simulink model "Y3Tiltrotor_sim3_INDI"  (R2025a)
settings: Solver=ode4  StartTime=0.0  StopTime=70  FixedStep=uavParam.sampleTime  RelTol=1e-3
PreLoadFcn:
  | filepath  = fileparts(get_param(bdroot, 'FileName'))
  | cd(filepath);
InitFcn:
  | Init_sim_INDI;
values from neighbouring files (symbols this model uses):
  control = struct    [Init_sim_INDI.m]
  env = struct    [InitData.m]
  flightState = struct    [Init_sim_INDI.m]
  FWSpeed0 = 15    [Init_sim_INDI.m]
  k_lpf_p = 50    [Init_sim_INDI.m]
  k_lpf_q = 80    [Init_sim_INDI.m]
  k_lpf_r = 5    [Init_sim_INDI.m]
  k_lpf_u = 10    [Init_sim_INDI.m]
  k_lpf_v = 1    [Init_sim_INDI.m]
  k_lpf_w = 50    [Init_sim_INDI.m]
  k_p = 5    [Init_sim_INDI.m]
  k_q = 20    [Init_sim_INDI.m]
  k_r = 1.5    [Init_sim_INDI.m]
  k_u = 0.5    [Init_sim_INDI.m]
  k_v = 0.5    [Init_sim_INDI.m]
  k_w = 2    [Init_sim_INDI.m]
  uavParam = struct    [InitData.m]
undefined symbols (not defined in the file or in its folder): ControlSampleTime, F, Light, MIL, Newton, Raphson
libraries: slpidlib x28, SignalEditorBlockLib x12, simulink x6, aerolibtransform2 x3, sharedtransform x3, robotcorelib x3, matrix_library x3, aerolibasang x2, aerolibutil x2, aerolibwind2 x2, shared6dof x1, aerolibatmos2 x1
(part 3 of 7)

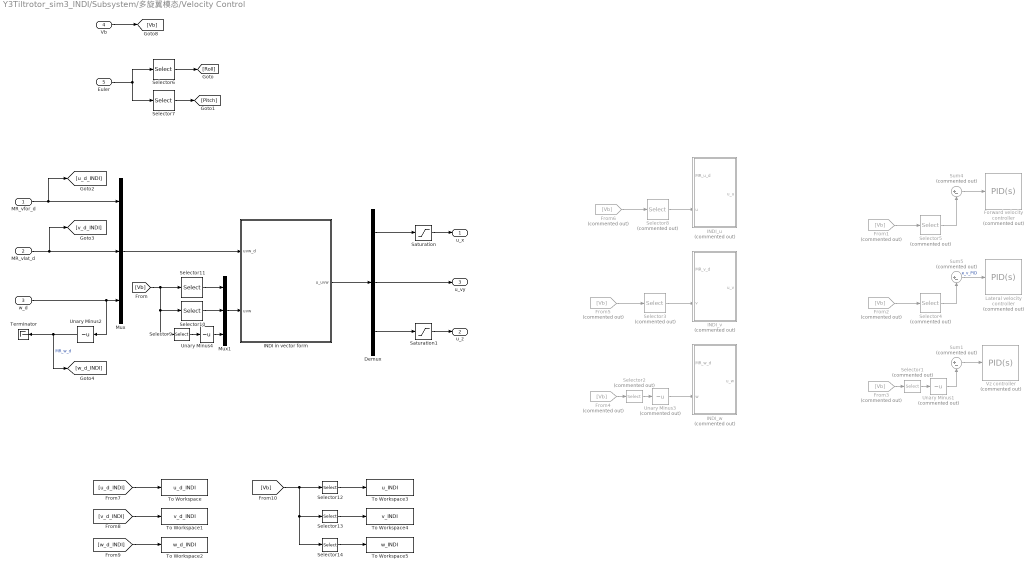
== system Y3Tiltrotor_sim3_INDI/Subsystem/多旋翼模态/Velocity Control ==
  MR_vfor_d : Inport
  MR_vlat_d : Inport  Port=2
  w_d : Inport  Port=3
  Vb : Inport  Port=4
  Euler : Inport  Port=5
  Demux : Demux  Outputs=3
  Forward velocity controller : slpidlib/PID Controller  Commented=on  Controller=PID  Form=Parallel  TimeDomain=Continuous-time  UseExternalTs=off  SampleTime=-1  IntegratorMethod=Forward Euler  FilterMethod=Forward Euler  ControllerParametersSource=internal  P=control.MR.vx_P  I=control.MR.vx_I  UseKiTs=off  D=control.MR.vx_D  UseExternalDerivativeSource=off  N=100  UseFilter=on  TunerSelectOption=Transfer Function Based (PID Tuner App)  InitialConditionSource=internal  InitialConditionForIntegrator=0  InitialConditionForFilter=0  DifferentiatorICPrevScaledInput=0  ExternalReset=none  TrackingMode=off  Kt=1  LimitOutput=off  SatLimitsSource=internal  UpperSaturationLimit=2  LowerSaturationLimit=-2  LinearizeAsGain=on  AntiWindupMode=none  Kb=1  LimitIntegrator=off  UpperIntegratorSaturationLimit=0.2  LowerIntegratorSaturationLimit=-0.2  POutMin=[]  POutMax=[]  IOutMin=[]  IOutMax=[]  DOutMin=[]  DOutMax=[]  NOutMin=[]  NOutMax=[]  SumOutMin=[]  SumOutMax=[]  SaturationOutMin=[]  SaturationOutMax=[]  PParamMin=[]  PParamMax=[]  IParamMin=[]  IParamMax=[]  DParamMin=[]  DParamMax=[]  NParamMin=[]  NParamMax=[]  KbParamMin=[]  KbParamMax=[]  KtParamMin=[]  KtParamMax=[]  KbOutMin=[]  KbOutMax=[]  KtOutMin=[]  KtOutMax=[]  IntegratorOutMin=[]  IntegratorOutMax=[]  FilterOutMin=[]  FilterOutMax=[]  SumI1OutMin=[]  SumI1OutMax=[]  SumI2OutMin=[]  SumI2OutMax=[]  SumI3OutMin=[]  SumI3OutMax=[]  SumI4OutMin=[]  SumI4OutMax=[]  SumDOutMin=[]  SumDOutMax=[]  DifferentiatorOutMin=[]  DifferentiatorOutMax=[]  FilterDiffOutCoefMin=[]  FilterDiffOutCoefMax=[]  ReciprocalOutMin=[]  ReciprocalOutMax=[]  SumDenOutMin=[]  SumDenOutMax=[]  SumNumOutMin=[]  SumNumOutMax=[]  DivideOutMin=[]  DivideOutMax=[]  UdiffTsProdOutMin=[]  UdiffTsProdOutMax=[]  NTsProdOutMin=[]  NTsProdOutMax=[]  UintegralTsProdOutMin=[]  UintegralTsProdOutMax=[]  UngainTsProdOutMin=[]  UngainTsProdOutMax=[]  ClampingZeroOutDataTypeStr=Inherit: Inherit via back propagation  ClampingZeroOutMin=[]  ClampingZeroOutMax=[]  FilterDenConstantOutDataTypeStr=Inherit: Inherit via back propagation  FilterDenConstantOutMin=[]  FilterDenConstantOutMax=[]  PCopyOutDataTypeStr=Inherit: Inherit via back propagation  PCopyOutMin=[]  PCopyOutMax=[]  NCopyOutDataTypeStr=Inherit: Inherit via back propagation  NCopyOutMin=[]  NCopyOutMax=[]  IntegratorContinuousStateAttributes=''  IntegratorStateMustResolveToSignalObject=off  IntegratorRTWStateStorageClass=Auto  FilterContinuousStateAttributes=''  FilterStateMustResolveToSignalObject=off  FilterRTWStateStorageClass=Auto  ParallelPVariant=InternalParameters  IdealPVariant=Disabled  IVariant=InternalParameters  DVariant=InternalParameters  IntegratorVariant=Continuous  SatVariant=Disabled  AWVariant=Passthrough  PCopyVariant=Disabled  TRVariant=Disabled  FdbkBlocksVariant=Forward  IdealPFdbkVariant=Disabled  SatFdbkVariant=Disabled  DerivativeFilterVariant=ContFilter  NVariant=InternalParameters  NCopyVariant=Disabled  FilterICVariant=InternalICsFilter  IntegratorICVariant=InternalICs  ExternalResetVariant=Disabled  TRSumVariant=Passthrough  SumFdbkVariant=Disabled  SumVariant=Sum_PID  TsampFilterVariant=InternalTs  TsampNgainVariant=Passthrough  TsampIntegralVariant=Disabled_SignalSpec  ExternalSaturationOutDataTypeStr=Inherit: Same as second input  DerivativeSourceVariant=ErrorSignal  PreIntVariant=InternalPreInt
  From{1..6} (6 alike) : From  Commented=on  GotoTag=Vb
  INDI in vector form : Subsystem
  INDI_u : Subsystem  Commented=on
  INDI_v : Subsystem  Commented=on
  INDI_w : Subsystem  Commented=on
  "Lateral velocity controller " : slpidlib/PID Controller  Commented=on  Controller=PID  Form=Parallel  TimeDomain=Continuous-time  UseExternalTs=off  SampleTime=-1  IntegratorMethod=Forward Euler  FilterMethod=Forward Euler  ControllerParametersSource=internal  P=control.MR.vy_P  I=control.MR.vy_I  UseKiTs=off  D=control.MR.vy_D  UseExternalDerivativeSource=off  N=100  UseFilter=on  TunerSelectOption=Transfer Function Based (PID Tuner App)  InitialConditionSource=internal  InitialConditionForIntegrator=0  InitialConditionForFilter=0  DifferentiatorICPrevScaledInput=0  ExternalReset=none  TrackingMode=off  Kt=1  LimitOutput=off  SatLimitsSource=internal  UpperSaturationLimit=control.maxRoll  LowerSaturationLimit=control.minRoll  LinearizeAsGain=on  AntiWindupMode=none  Kb=1  LimitIntegrator=off  UpperIntegratorSaturationLimit=inf  LowerIntegratorSaturationLimit=-inf  POutMin=[]  POutMax=[]  IOutMin=[]  IOutMax=[]  DOutMin=[]  DOutMax=[]  NOutMin=[]  NOutMax=[]  SumOutMin=[]  SumOutMax=[]  SaturationOutMin=[]  SaturationOutMax=[]  PParamMin=[]  PParamMax=[]  IParamMin=[]  IParamMax=[]  DParamMin=[]  DParamMax=[]  NParamMin=[]  NParamMax=[]  KbParamMin=[]  KbParamMax=[]  KtParamMin=[]  KtParamMax=[]  KbOutMin=[]  KbOutMax=[]  KtOutMin=[]  KtOutMax=[]  IntegratorOutMin=[]  IntegratorOutMax=[]  FilterOutMin=[]  FilterOutMax=[]  SumI1OutMin=[]  SumI1OutMax=[]  SumI2OutMin=[]  SumI2OutMax=[]  SumI3OutMin=[]  SumI3OutMax=[]  SumI4OutMin=[]  SumI4OutMax=[]  SumDOutMin=[]  SumDOutMax=[]  DifferentiatorOutMin=[]  DifferentiatorOutMax=[]  FilterDiffOutCoefMin=[]  FilterDiffOutCoefMax=[]  ReciprocalOutMin=[]  ReciprocalOutMax=[]  SumDenOutMin=[]  SumDenOutMax=[]  SumNumOutMin=[]  SumNumOutMax=[]  DivideOutMin=[]  DivideOutMax=[]  UdiffTsProdOutMin=[]  UdiffTsProdOutMax=[]  NTsProdOutMin=[]  NTsProdOutMax=[]  UintegralTsProdOutMin=[]  UintegralTsProdOutMax=[]  UngainTsProdOutMin=[]  UngainTsProdOutMax=[]  ClampingZeroOutDataTypeStr=Inherit: Inherit via back propagation  ClampingZeroOutMin=[]  ClampingZeroOutMax=[]  FilterDenConstantOutDataTypeStr=Inherit: Inherit via back propagation  FilterDenConstantOutMin=[]  FilterDenConstantOutMax=[]  PCopyOutDataTypeStr=Inherit: Inherit via back propagation  PCopyOutMin=[]  PCopyOutMax=[]  NCopyOutDataTypeStr=Inherit: Inherit via back propagation  NCopyOutMin=[]  NCopyOutMax=[]  IntegratorContinuousStateAttributes=''  IntegratorStateMustResolveToSignalObject=off  IntegratorRTWStateStorageClass=Auto  FilterContinuousStateAttributes=''  FilterStateMustResolveToSignalObject=off  FilterRTWStateStorageClass=Auto  ParallelPVariant=InternalParameters  IdealPVariant=Disabled  IVariant=InternalParameters  DVariant=InternalParameters  IntegratorVariant=Continuous  SatVariant=Disabled  AWVariant=Passthrough  PCopyVariant=Disabled  TRVariant=Disabled  FdbkBlocksVariant=Forward  IdealPFdbkVariant=Disabled  SatFdbkVariant=Disabled  DerivativeFilterVariant=ContFilter  NVariant=InternalParameters  NCopyVariant=Disabled  FilterICVariant=InternalICsFilter  IntegratorICVariant=InternalICs  ExternalResetVariant=Disabled  TRSumVariant=Passthrough  SumFdbkVariant=Disabled  SumVariant=Sum_PID  TsampFilterVariant=InternalTs  TsampNgainVariant=Passthrough  TsampIntegralVariant=Disabled_SignalSpec  ExternalSaturationOutDataTypeStr=Inherit: Same as second input  DerivativeSourceVariant=ErrorSignal  PreIntVariant=InternalPreInt
  Mux : Mux  Inputs=3
  Mux1 : Mux  Inputs=3
  Saturation : Saturate  UpperLimit=2  LowerLimit=-2
  Saturation1 : Saturate  UpperLimit=3  LowerLimit=0
  Selector1 : Selector  Commented=on  InputPortWidth=3  IndexOptions=Index vector (dialog)  Indices=3  OutputSizes=1
  Selector10 : Selector  InputPortWidth=3  IndexOptions=Index vector (dialog)  Indices=2  OutputSizes=1
  Selector11 : Selector  InputPortWidth=3  IndexOptions=Index vector (dialog)  Indices=1  OutputSizes=1
  Selector12 : Selector  InputPortWidth=3  IndexOptions=Index vector (dialog)  Indices=1  OutputSizes=1
  Selector13 : Selector  InputPortWidth=3  IndexOptions=Index vector (dialog)  Indices=2  OutputSizes=1
  Selector14 : Selector  InputPortWidth=3  IndexOptions=Index vector (dialog)  Indices=3  OutputSizes=1
  Selector2 : Selector  Commented=on  InputPortWidth=3  IndexOptions=Index vector (dialog)  Indices=3  OutputSizes=1
  Selector3 : Selector  Commented=on  InputPortWidth=3  IndexOptions=Index vector (dialog)  Indices=2  OutputSizes=1
  Selector4 : Selector  Commented=on  InputPortWidth=3  IndexOptions=Index vector (dialog)  Indices=2  OutputSizes=1
  Selector5 : Selector  Commented=on  InputPortWidth=3  IndexOptions=Index vector (dialog)  Indices=1  OutputSizes=1
  Selector6 : Selector  InputPortWidth=3  IndexOptions=Index vector (dialog)  Indices=1  OutputSizes=1
  Selector7 : Selector  InputPortWidth=3  IndexOptions=Index vector (dialog)  Indices=2  OutputSizes=1
  Selector8 : Selector  Commented=on  InputPortWidth=3  IndexOptions=Index vector (dialog)  Indices=1  OutputSizes=1
  Selector9 : Selector  InputPortWidth=3  IndexOptions=Index vector (dialog)  Indices=3  OutputSizes=1
  Sum1 : Sum  Commented=on  Inputs=|+-
  Sum4 : Sum  Commented=on  Inputs=|+-
  Sum5 : Sum  Commented=on  Inputs=|+-
  Terminator : Terminator
  To Workspace : ToWorkspace  VariableName=u_d_INDI  SampleTime=-1
      settings: Save2DSignal=2-D array (concatenate along first dimension)
  To Workspace1 : ToWorkspace  VariableName=v_d_INDI  SampleTime=-1
      settings: Save2DSignal=2-D array (concatenate along first dimension)
  To Workspace2 : ToWorkspace  VariableName=w_d_INDI  SampleTime=-1
      settings: Save2DSignal=2-D array (concatenate along first dimension)
  To Workspace3 : ToWorkspace  VariableName=u_INDI  SampleTime=-1
      settings: Save2DSignal=2-D array (concatenate along first dimension)
  To Workspace4 : ToWorkspace  VariableName=v_INDI  SampleTime=-1
      settings: Save2DSignal=2-D array (concatenate along first dimension)
  To Workspace5 : ToWorkspace  VariableName=w_INDI  SampleTime=-1
      settings: Save2DSignal=2-D array (concatenate along first dimension)
  Unary Minus1 : UnaryMinus  Commented=on
  Unary Minus2 : UnaryMinus
  Unary Minus3 : UnaryMinus  Commented=on
  Unary Minus4 : UnaryMinus
  Vz controller : slpidlib/PID Controller  Commented=on  Controller=PID  Form=Parallel  TimeDomain=Continuous-time  UseExternalTs=off  SampleTime=ControlSampleTime  IntegratorMethod=Forward Euler  FilterMethod=Forward Euler  ControllerParametersSource=internal  P=control.MR.vz_P  I=control.MR.vz_I  UseKiTs=off  D=control.MR.vz_D  UseExternalDerivativeSource=off  N=100  UseFilter=on  TunerSelectOption=Transfer Function Based (PID Tuner App)  InitialConditionSource=internal  InitialConditionForIntegrator=0  InitialConditionForFilter=0  DifferentiatorICPrevScaledInput=0  ExternalReset=none  TrackingMode=off  Kt=1  LimitOutput=off  SatLimitsSource=internal  UpperSaturationLimit=3  LowerSaturationLimit=0  LinearizeAsGain=on  AntiWindupMode=clamping  Kb=1  LimitIntegrator=off  UpperIntegratorSaturationLimit=inf  LowerIntegratorSaturationLimit=-inf  POutMin=[]  POutMax=[]  IOutMin=[]  IOutMax=[]  DOutMin=[]  DOutMax=[]  NOutMin=[]  NOutMax=[]  SumOutMin=[]  SumOutMax=[]  SaturationOutMin=[]  SaturationOutMax=[]  PParamMin=[]  PParamMax=[]  IParamMin=[]  IParamMax=[]  DParamMin=[]  DParamMax=[]  NParamMin=[]  NParamMax=[]  KbParamMin=[]  KbParamMax=[]  KtParamMin=[]  KtParamMax=[]  KbOutMin=[]  KbOutMax=[]  KtOutMin=[]  KtOutMax=[]  IntegratorOutMin=[]  IntegratorOutMax=[]  FilterOutMin=[]  FilterOutMax=[]  SumI1OutMin=[]  SumI1OutMax=[]  SumI2OutMin=[]  SumI2OutMax=[]  SumI3OutMin=[]  SumI3OutMax=[]  SumI4OutMin=[]  SumI4OutMax=[]  SumDOutMin=[]  SumDOutMax=[]  DifferentiatorOutMin=[]  DifferentiatorOutMax=[]  FilterDiffOutCoefMin=[]  FilterDiffOutCoefMax=[]  ReciprocalOutMin=[]  ReciprocalOutMax=[]  SumDenOutMin=[]  SumDenOutMax=[]  SumNumOutMin=[]  SumNumOutMax=[]  DivideOutMin=[]  DivideOutMax=[]  UdiffTsProdOutMin=[]  UdiffTsProdOutMax=[]  NTsProdOutMin=[]  NTsProdOutMax=[]  UintegralTsProdOutMin=[]  UintegralTsProdOutMax=[]  UngainTsProdOutMin=[]  UngainTsProdOutMax=[]  ClampingZeroOutDataTypeStr=Inherit: Inherit via back propagation  ClampingZeroOutMin=[]  ClampingZeroOutMax=[]  FilterDenConstantOutDataTypeStr=Inherit: Inherit via back propagation  FilterDenConstantOutMin=[]  FilterDenConstantOutMax=[]  PCopyOutDataTypeStr=Inherit: Inherit via back propagation  PCopyOutMin=[]  PCopyOutMax=[]  NCopyOutDataTypeStr=Inherit: Inherit via back propagation  NCopyOutMin=[]  NCopyOutMax=[]  IntegratorContinuousStateAttributes=''  IntegratorStateMustResolveToSignalObject=off  IntegratorRTWStateStorageClass=Auto  FilterContinuousStateAttributes=''  FilterStateMustResolveToSignalObject=off  FilterRTWStateStorageClass=Auto  ParallelPVariant=InternalParameters  IdealPVariant=Disabled  IVariant=InternalParameters  DVariant=InternalParameters  IntegratorVariant=Continuous  SatVariant=Disabled  AWVariant=Passthrough  PCopyVariant=Disabled  TRVariant=Disabled  FdbkBlocksVariant=Forward  IdealPFdbkVariant=Disabled  SatFdbkVariant=Disabled  DerivativeFilterVariant=ContFilter  NVariant=InternalParameters  NCopyVariant=Disabled  FilterICVariant=InternalICsFilter  IntegratorICVariant=InternalICs  ExternalResetVariant=Disabled  TRSumVariant=Passthrough  SumFdbkVariant=Disabled  SumVariant=Sum_PID  TsampFilterVariant=InternalTs  TsampNgainVariant=Passthrough  TsampIntegralVariant=Disabled_SignalSpec  ExternalSaturationOutDataTypeStr=Inherit: Same as second input  DerivativeSourceVariant=ErrorSignal  PreIntVariant=InternalPreInt
  u_x : Outport
  u_z : Outport  Port=2
  u_vy : Outport  Port=3
  wires:
  Unary Minus1/1 -> Sum1/2
  Selector1/1 -> Unary Minus1/1
  Vb/1 -> [Vb]
  From3/1 -> Selector1/1
  w_d/1 -> Mux/3, Unary Minus2/1
  Sum1/1 -> Vz controller/1
  Euler/1 -> Selector6/1, Selector7/1
  Selector7/1 -> [Pitch]
  Selector6/1 -> [Roll]
  Saturation/1 -> u_x/1
  Saturation1/1 -> u_z/1
  Unary Minus2/1 -> [w_d_INDI], Terminator/1  "MR_w_d"
  Selector4/1 -> Sum5/2
  From2/1 -> Selector4/1
  Sum5/1 -> "Lateral velocity controller "/1  "e_v_PID"
  Sum4/1 -> Forward velocity controller/1
  From1/1 -> Selector5/1
  Selector5/1 -> Sum4/2
  INDI in vector form/1(u_uvw) -> Demux/1
  Mux1/1 -> INDI in vector form/2(uvw)
  Mux/1 -> INDI in vector form/1(uvw_d)
  From6/1 -> Selector8/1
  Selector8/1 -> INDI_u/2(u)
  Selector3/1 -> INDI_v/2(v)
  From5/1 -> Selector3/1
  Unary Minus3/1 -> INDI_w/2(w)
  Selector2/1 -> Unary Minus3/1
  From4/1 -> Selector2/1
  MR_vfor_d/1 -> [u_d_INDI], Mux/1
  MR_vlat_d/1 -> [v_d_INDI], Mux/2
  Selector9/1 -> Unary Minus4/1
  [Vb] -> Selector11/1, Selector10/1, Selector9/1
  Selector11/1 -> Mux1/1
  Selector10/1 -> Mux1/2
  Unary Minus4/1 -> Mux1/3
  Demux/1 -> Saturation/1
  Demux/2 -> u_vy/1
  Demux/3 -> Saturation1/1
  [u_d_INDI] -> To Workspace/1
  [v_d_INDI] -> To Workspace1/1
  [w_d_INDI] -> To Workspace2/1
  [Vb] -> Selector13/1, Selector14/1, Selector12/1
  Selector12/1 -> To Workspace3/1
  Selector13/1 -> To Workspace4/1
  Selector14/1 -> To Workspace5/1

== system Y3Tiltrotor_sim3_INDI/Subsystem/混控器/固定翼混控 ==
  FlightMode : Inport
  "FixedwingControlOutput " : Inport  Port=2
  Merge : Merge  Inputs=4
  Switch Case : SwitchCase  CaseConditions={flightState.Hover, flightState.Transition, flightState.FixedWing,flightState.BackTransition}  ShowDefaultCase=off
  固定翼模态混控 : Subsystem
  旋翼模态混控 : Subsystem
  toMultirotorMixer : Outport
  FixedwingCtrlSurface : Outport  Port=2
  wires:
  "FixedwingControlOutput "/1 -> 固定翼模态混控/1("FixedwingControlOutput ")
  固定翼模态混控/1(toMultirotorMixer) -> toMultirotorMixer/1
  FlightMode/1 -> Switch Case/1
  Merge/1 -> FixedwingCtrlSurface/1
  固定翼模态混控/2(FixedwingCtrlSurface) -> Merge/3
  Switch Case/3 -> 固定翼模态混控/Action
  旋翼模态混控/1(FixedwingCtrlSurface) -> Merge/1
  Switch Case/1 -> 旋翼模态混控/Action

== system Y3Tiltrotor_sim3_INDI/Subsystem/混控器/多旋翼混控 ==
  States : Inport
  "MultirotorControlOutput " : Inport  Port=2
  FlightMode : Inport  Port=3
  toMultirotorMixer : Inport  Port=4
  Actuator To Voltage : Subsystem
  Merge : Merge  Inputs=4
  Switch Case : SwitchCase  CaseConditions={flightState.Hover, flightState.Transition, flightState.FixedWing,flightState.BackTransition}  ShowDefaultCase=off
  固定翼模态混控 : Subsystem
  旋翼模态混控 : Subsystem
  MultirotorActuator : Outport
  wires:
  toMultirotorMixer/1 -> 固定翼模态混控/1(toMultirotorMixer)
  固定翼模态混控/1(MultirotorActuator) -> Merge/3
  FlightMode/1 -> Switch Case/1
  Switch Case/3 -> 固定翼模态混控/Action
  Switch Case/1 -> 旋翼模态混控/Action
  "MultirotorControlOutput "/1 -> 旋翼模态混控/1("MultirotorControlOutput ")
  旋翼模态混控/1(MultirotorActuator) -> Merge/1
  Actuator To Voltage/1(To PWM) -> MultirotorActuator/1
  Merge/1 -> Actuator To Voltage/1(Motor Commands)
  States/1 -> 旋翼模态混控/2(states)

== system Y3Tiltrotor_sim3_INDI/Y3 Tiltrotor Aircraft Model/Subsystem/Aerodynamic Forces and Moments ==
  note: FIMI Manta飞行器气动力和力矩的计算需要参考飞翼布局的飞行器，它只有升降副翼，没有尾翼。
  CtrlSurfaces : Inport
  Wind_e : Inport  Port=2
  UAV State : Inport  Port=3
  Bus Selector2 : BusSelector  OutputSignals=DCMbe,Ve,Xe
  Compute Air Data : Subsystem  TreatAsAtomicUnit=on  VariantControl=use_aerospace_blocks == 1
  Compute Body Frame Aerodynamic Forces and Moments : Subsystem
  Compute Rho : Subsystem
  RL2B * Vw : Product  Multiplication=Matrix(*)  InputSameDT=on  SaturateOnIntegerOverflow=on  OutDataTypeStr=Inherit: Same as first input
  Vair : Sum  Inputs=+-  InputSameDT=on  SaturateOnIntegerOverflow=on  OutDataTypeStr=Inherit: Same as first input
  AirData : Outport  VectorParamsAs1DForOutWhenUnconnected=off
  F_aero : Outport  Port=2  VectorParamsAs1DForOutWhenUnconnected=off
  M_aero : Outport  Port=3  VectorParamsAs1DForOutWhenUnconnected=off
  wires:
  Bus Selector2/2 -> Vair/1  "<Ve>"
  UAV State/1 -> Bus Selector2/1
  Wind_e/1 -> Vair/2
  Compute Air Data/1(AirData) -> AirData/1, Compute Body Frame Aerodynamic Forces and Moments/1(AirData)
  RL2B * Vw/1 -> Compute Air Data/1(Vb)
  Compute Rho/1(Rho) -> Compute Air Data/2(Rho)
  Vair/1 -> RL2B * Vw/2
  Bus Selector2/3 -> Compute Rho/1(Xe)  "<Xe>"
  Bus Selector2/1 -> RL2B * Vw/1  "<DCMbe>"
  CtrlSurfaces/1 -> Compute Body Frame Aerodynamic Forces and Moments/2(CtrlSurfaces)
  Compute Body Frame Aerodynamic Forces and Moments/1(F_b) -> F_aero/1
  Compute Body Frame Aerodynamic Forces and Moments/2(M_b) -> M_aero/1

== system Y3Tiltrotor_sim3_INDI/Y3 Tiltrotor Aircraft Model/Subsystem/Gravity ==
  DCM_be : Inport
  Constant : Constant  Value=[0 0 uavParam.aero.g]'
  Gain : Gain  Gain=uavParam.geom.mass
  Matrix Multiply : Product  Multiplication=Matrix(*)
  F_g : Outport
  wires:
  Matrix Multiply/1 -> Gain/1
  Constant/1 -> Matrix Multiply/2
  DCM_be/1 -> Matrix Multiply/1
  Gain/1 -> F_g/1

== system Y3Tiltrotor_sim3_INDI/Y3 Tiltrotor Aircraft Model/Subsystem/GroundModel1 ==
  UavState : Inport
  "TerrainZ " : Inport  Port=2
  Bus Selector : BusSelector  OutputSignals=pqr,Xe,Ve,Euler,DCMbe
  Direction Cosine Matrix to Quaternions : sharedtransform/Direction Cosine Matrix  to Quaternions  aMode=aMode  action=None  tolerance=eps(2)
  Direction Cosine Matrix to Quaternions1 : sharedtransform/Direction Cosine Matrix  to Quaternions  aMode=aMode  action=None  tolerance=eps(2)
  Euler to DCM : aerolibtransform2/Wind Angles to  Direction Cosine Matrix
  Gain : Gain  Gain=[0 0 9.8]
  Ground Model New : Subsystem
  ModelParam.uavMass : Constant  Value=uavParam.geom.mass
  OnGroundFaceup : Subsystem
  Product : Product  Multiplication=Matrix(*)
  Quaternion Inverse : aerolibutil/Quaternion Inverse
  Quaternion Multiplication : aerolibutil/Quaternion Multiplication
  F_Ground : Outport  VectorParamsAs1DForOutWhenUnconnected=off
  M_Ground : Outport  Port=2  VectorParamsAs1DForOutWhenUnconnected=off
  wires:
  "TerrainZ "/1 -> Ground Model New/6(TerrainZ)
  Ground Model New/2(M1) -> M_Ground/1  "Mb"
  Product/1 -> F_Ground/1  "Fb"
  Quaternion Multiplication/1 -> Ground Model New/5(Quet)
  Quaternion Inverse/1 -> Quaternion Multiplication/1
  Direction Cosine Matrix to Quaternions1/1 -> Quaternion Inverse/1
  Euler to DCM/1 -> Direction Cosine Matrix to Quaternions1/1
  OnGroundFaceup/1(y) -> Euler to DCM/1
  Direction Cosine Matrix to Quaternions/1 -> Quaternion Multiplication/2
  Ground Model New/1(F1) -> Product/2
  UavState/1 -> Bus Selector/1
  ModelParam.uavMass/1 -> Gain/1
  Gain/1 -> Ground Model New/1(mg)
  Bus Selector/5 -> Product/1, Direction Cosine Matrix to Quaternions/1  "<DCMbe>"
  Bus Selector/4 -> OnGroundFaceup/1(Eular(rad))  "<Euler>"
  Bus Selector/3 -> Ground Model New/4(Ve)  "<Ve>"
  Bus Selector/2 -> Ground Model New/3(Xe)  "<Xe>"
  Bus Selector/1 -> Ground Model New/2(wb)  "<pqr>"

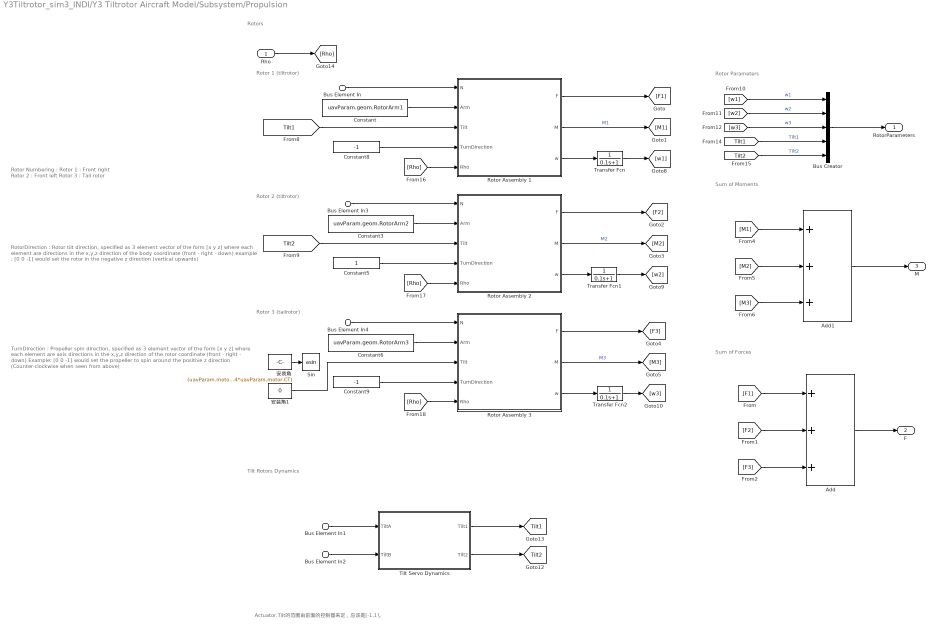
== system Y3Tiltrotor_sim3_INDI/Y3 Tiltrotor Aircraft Model/Subsystem/Propulsion ==
  note: Actuator.Tilt的范围由前面的控制器来定，应该是[-1,1]。
  note: TurnDirection : Propeller spin direction, specified as 3 element vector of the form [x y z] where each element are axis directions in the x,y,z direction of the rotor coordinate (front - right - down)
      |
      | Example: [0 0 -1] would set the propeller to spin around the positive z direction (Counter-clockwise when seen from above)
  note: RotorDirection : Rotor tilt direction, specified as 3 element vector of the form [x y z] where each element are directions in the x,y,z direction of the body coordinate (front - right - down)
      |
      | example : [0 0 -1] would set the rotor in the negative z direction (vertical upwards)
  note: Rotor Numbering :
      | Rotor 1 : Front right
      | Rotor 2 : Front left
      | Rotor 3 : Tail rotor
  note: Tilt Rotors Dynamics
  note: Sum of Moments
  note: Rotor 1
      | (tiltrotor)
  note: Rotors
  note: Rotor 2
      | (tiltrotor)
  note: Rotor 3
      | (tailrotor)
  note: Sum of Forces
  note: Rotor Parameters
  Rho : Inport
  Bus Element In : Inport  Port=2  PortName=Actuator  Element=w1
  Bus Element In1 : Inport  Port=2  PortName=Actuator  Element=Tilt1
  Bus Element In2 : Inport  Port=2  PortName=Actuator  Element=Tilt2
  Bus Element In3 : Inport  Port=2  PortName=Actuator  Element=w2
  Bus Element In4 : Inport  Port=2  PortName=Actuator  Element=w3
  Add : Sum  Inputs=+++
  Add1 : Sum  Inputs=+++
  Bus Creator : BusCreator  Inputs=5
  Constant : Constant  Value=uavParam.geom.RotorArm1
  Constant3 : Constant  Value=uavParam.geom.RotorArm2
  Constant5 : Constant
  Constant6 : Constant  Value=uavParam.geom.RotorArm3
  Constant8 : Constant  Value=-1
  Constant9 : Constant  Value=-1
  Rotor Assembly 1 : Subsystem
  Rotor Assembly 2 : Subsystem
  "Rotor Assembly 3 " : Subsystem
  Sin : Trigonometry  Operator=asin
  Tilt Servo Dynamics : Subsystem
  Transfer Fcn : TransferFcn  Denominator=[0.1 1]
  Transfer Fcn1 : TransferFcn  Denominator=[0.1 1]
  Transfer Fcn2 : TransferFcn  Denominator=[0.1 1]
  安装角 : Constant  Value=(uavParam.motor.CQ*uavParam.geom.PropRadius)/(0.24*uavParam.motor.CT)
  安装角1 : Constant  Value=0
  RotorParameters : Outport
  F : Outport  Port=2
  M : Outport  Port=3
  tag scope: Tilt1=global, Tilt2=global
  wires:
  Constant/1 -> Rotor Assembly 1/2(Arm)
  [Tilt1] -> Rotor Assembly 1/3(Tilt)
  Add/1 -> F/1
  Constant8/1 -> Rotor Assembly 1/4(TurnDirection)
  Rotor Assembly 1/1(F) -> [F1]
  Rotor Assembly 1/2(M) -> [M1]  "M1"
  Rotor Assembly 2/1(F) -> [F2]
  Constant3/1 -> Rotor Assembly 2/2(Arm)
  Constant5/1 -> Rotor Assembly 2/4(TurnDirection)
  Rotor Assembly 2/2(M) -> [M2]  "M2"
  "Rotor Assembly 3 "/1(F) -> [F3]
  Constant6/1 -> "Rotor Assembly 3 "/2(Arm)
  Constant9/1 -> "Rotor Assembly 3 "/4(TurnDirection)
  安装角/1 -> Sin/1
  "Rotor Assembly 3 "/2(M) -> [M3]  "M3"
  [F1] -> Add/1
  [F2] -> Add/2
  [F3] -> Add/3
  Add1/1 -> M/1
  [M3] -> Add1/3
  [M2] -> Add1/2
  [M1] -> Add1/1
  Rotor Assembly 1/3(w) -> Transfer Fcn/1
  Rotor Assembly 2/3(w) -> Transfer Fcn1/1
  "Rotor Assembly 3 "/3(w) -> Transfer Fcn2/1
  [w1] -> Bus Creator/1  "w1"
  [w2] -> Bus Creator/2  "w2"
  [w3] -> Bus Creator/3  "w3"
  Bus Creator/1 -> RotorParameters/1
  [Tilt1] -> Bus Creator/4  "Tilt1"
  [Tilt2] -> Bus Creator/5  "Tilt2"
  Bus Element In/1 -> Rotor Assembly 1/1(N)
  Bus Element In3/1 -> Rotor Assembly 2/1(N)
  Bus Element In4/1 -> "Rotor Assembly 3 "/1(N)
  Tilt Servo Dynamics/1(Tilt1) -> [Tilt1]
  Tilt Servo Dynamics/2(Tilt2) -> [Tilt2]
  Bus Element In1/1 -> Tilt Servo Dynamics/1(TiltA)
  Bus Element In2/1 -> Tilt Servo Dynamics/2(TiltB)
  Transfer Fcn/1 -> [w1]
  Transfer Fcn1/1 -> [w2]
  Transfer Fcn2/1 -> [w3]
  Rho/1 -> [Rho]
  [Rho] -> Rotor Assembly 1/5(Rho)
  [Tilt2] -> Rotor Assembly 2/3(Tilt)
  [Rho] -> Rotor Assembly 2/5(Rho)
  [Rho] -> "Rotor Assembly 3 "/5(Rho)
  安装角1/1 -> "Rotor Assembly 3 "/3(Tilt)

== system Y3Tiltrotor_sim3_INDI/Y3 Tiltrotor Aircraft Model/Subsystem/Weather Model_org ==
  UavState : Inport
  if Wind On : Inport  Port=2
  " Compute Norm" : Subsystem
  Add : Sum  Inputs=2
  Bus Selector : BusSelector  OutputSignals=Euler,Xe,Ve
  Constant : Constant  Value=[0 0 0]
      settings: AttributesFormatString=%<Value>
  Dryden Wind Turbulence Model : aerolibwind2/Dryden Wind Turbulence Model  (Continuous (+q -r))  units=Metric (MKS)  spec=MIL-F-8785C  model=Continuous Dryden (+q -r)  W20=env.windBase/4  Wdeg=env.windDirTurb  TurbProb=10^-2 - Light  L_high=533.4  Wingspan=uavParam.geom.span  ts=ap.apSampleTime  Seed=[23341 23342 23343 23344]  T_on=on
  Gain1 : Gain  Gain=-1
      settings: AttributesFormatString=Z to Alt
  Get Z1 : Selector  InputPortWidth=3  IndexOptions=Index vector (dialog)  Indices=[3]  OutputSizes=[(-2)]
  "Horizontal Wind Model " : aerolibwind2/Horizontal Wind Model  units=Metric (MKS)  Vw_source=Internal  Vwind=env.windBase  W_source=Internal  Wdeg=env.windDirHor
  RL2B : Subsystem
  Reduce Z Wind : Gain  Gain=[1 1 0.1]
      settings: AttributesFormatString=%<Gain>
  Rotate to E Frame : Product  Multiplication=Matrix(*)
  Switch : Switch  Criteria=u2 > Threshold  Threshold=0.3  SaturateOnIntegerOverflow=off  InputSameDT=off
  Terminator : Terminator
  Transpose : Math  Operator=transpose  SignedPower=on
  "[0, pi] Wrap Around" : Subsystem
  Wind_e : Outport  Unit=m/s  VectorParamsAs1DForOutWhenUnconnected=off
  wires:
  Bus Selector/1 -> "[0, pi] Wrap Around"/1(Euler)  "<Euler>"
  Dryden Wind Turbulence Model/2 -> Terminator/1
  Constant/1 -> Switch/3
  Get Z1/1 -> Gain1/1
  RL2B/1(RL2B) -> "Horizontal Wind Model "/1, Dryden Wind Turbulence Model/3, Transpose/1  "RECEF2B"
  Transpose/1 -> Rotate to E Frame/1
  Rotate to E Frame/1 -> Wind_e/1
  Switch/1 -> Rotate to E Frame/2
  Dryden Wind Turbulence Model/1 -> Reduce Z Wind/1
  " Compute Norm"/1(V) -> Dryden Wind Turbulence Model/2
  Gain1/1 -> Dryden Wind Turbulence Model/1
  "Horizontal Wind Model "/1 -> Add/2
  Reduce Z Wind/1 -> Add/1
  Add/1 -> Switch/1
  if Wind On/1 -> Switch/2
  "[0, pi] Wrap Around"/1(Wrapped) -> RL2B/1(Euler)  "Euler"
  UavState/1 -> Bus Selector/1
  Bus Selector/3 -> " Compute Norm"/1(<Ve>)  "<Ve>"
  Bus Selector/2 -> Get Z1/1  "<Xe>"

== system Y3Tiltrotor_sim3_INDI/Subsystem/固定翼模态/attitude control/Turn Coordinator ==
  Roll SP : Inport
  Pitch SP : Inport  Port=2
  Airspeed : Inport  Port=3
  r : Inport  Port=4
  MATLAB Function : MATLAB Function  TreatAsAtomicUnit=on
  Sum : Sum  Inputs=|+-
  YawRate Controller : slpidlib/PID Controller  Controller=PID  Form=Parallel  TimeDomain=Discrete-time  UseExternalTs=off  SampleTime=-1  IntegratorMethod=Forward Euler  FilterMethod=Forward Euler  ControllerParametersSource=internal  P=control.FW.yawRate_P  I=control.FW.yawRate_I  UseKiTs=off  D=control.FW.yawRate_D  UseExternalDerivativeSource=off  N=100  UseFilter=on  TunerSelectOption=Transfer Function Based (PID Tuner App)  InitialConditionSource=internal  InitialConditionForIntegrator=0  InitialConditionForFilter=0  DifferentiatorICPrevScaledInput=0  ExternalReset=none  TrackingMode=off  Kt=1  LimitOutput=on  SatLimitsSource=internal  UpperSaturationLimit=1  LowerSaturationLimit=-1  LinearizeAsGain=on  AntiWindupMode=none  Kb=1  LimitIntegrator=off  UpperIntegratorSaturationLimit=inf  LowerIntegratorSaturationLimit=-inf  POutMin=[]  POutMax=[]  IOutMin=[]  IOutMax=[]  DOutMin=[]  DOutMax=[]  NOutMin=[]  NOutMax=[]  SumOutMin=[]  SumOutMax=[]  SaturationOutMin=[]  SaturationOutMax=[]  PParamMin=[]  PParamMax=[]  IParamMin=[]  IParamMax=[]  DParamMin=[]  DParamMax=[]  NParamMin=[]  NParamMax=[]  KbParamMin=[]  KbParamMax=[]  KtParamMin=[]  KtParamMax=[]  KbOutMin=[]  KbOutMax=[]  KtOutMin=[]  KtOutMax=[]  IntegratorOutMin=[]  IntegratorOutMax=[]  FilterOutMin=[]  FilterOutMax=[]  SumI1OutMin=[]  SumI1OutMax=[]  SumI2OutMin=[]  SumI2OutMax=[]  SumI3OutMin=[]  SumI3OutMax=[]  SumI4OutMin=[]  SumI4OutMax=[]  SumDOutMin=[]  SumDOutMax=[]  DifferentiatorOutMin=[]  DifferentiatorOutMax=[]  FilterDiffOutCoefMin=[]  FilterDiffOutCoefMax=[]  ReciprocalOutMin=[]  ReciprocalOutMax=[]  SumDenOutMin=[]  SumDenOutMax=[]  SumNumOutMin=[]  SumNumOutMax=[]  DivideOutMin=[]  DivideOutMax=[]  UdiffTsProdOutMin=[]  UdiffTsProdOutMax=[]  NTsProdOutMin=[]  NTsProdOutMax=[]  UintegralTsProdOutMin=[]  UintegralTsProdOutMax=[]  UngainTsProdOutMin=[]  UngainTsProdOutMax=[]  ClampingZeroOutDataTypeStr=Inherit: Inherit via back propagation  ClampingZeroOutMin=[]  ClampingZeroOutMax=[]  FilterDenConstantOutDataTypeStr=Inherit: Inherit via back propagation  FilterDenConstantOutMin=[]  FilterDenConstantOutMax=[]  PCopyOutDataTypeStr=Inherit: Inherit via back propagation  PCopyOutMin=[]  PCopyOutMax=[]  NCopyOutDataTypeStr=Inherit: Inherit via back propagation  NCopyOutMin=[]  NCopyOutMax=[]  IntegratorContinuousStateAttributes=''  IntegratorStateMustResolveToSignalObject=off  IntegratorRTWStateStorageClass=Auto  FilterContinuousStateAttributes=''  FilterStateMustResolveToSignalObject=off  FilterRTWStateStorageClass=Auto  ParallelPVariant=InternalParameters  IdealPVariant=Disabled  IVariant=InternalParameters  DVariant=InternalParameters  IntegratorVariant=Discrete  SatVariant=Enabled  AWVariant=Passthrough  PCopyVariant=Disabled  TRVariant=Disabled  FdbkBlocksVariant=Forward  IdealPFdbkVariant=Disabled  SatFdbkVariant=Disabled  DerivativeFilterVariant=ForwardEulerFilter  NVariant=InternalParameters  NCopyVariant=Disabled  FilterICVariant=InternalICsFilter  IntegratorICVariant=InternalICs  ExternalResetVariant=Disabled  TRSumVariant=Passthrough  SumFdbkVariant=Disabled  SumVariant=Sum_PID  TsampFilterVariant=InternalTs  TsampNgainVariant=Passthrough  TsampIntegralVariant=Disabled_SignalSpec  ExternalSaturationOutDataTypeStr=Inherit: Same as second input  DerivativeSourceVariant=ErrorSignal  PreIntVariant=InternalPreInt
  Tau_z : Outport
  wires:
  Roll SP/1 -> MATLAB Function/1(rollSP)
  Pitch SP/1 -> MATLAB Function/2(pitchSP)
  Airspeed/1 -> MATLAB Function/3(airSpeed)
  Sum/1 -> YawRate Controller/1
  YawRate Controller/1 -> Tau_z/1  "Tau_z"
  r/1 -> Sum/2  "r"
  MATLAB Function/1(rSP) -> Sum/1  "FW_r_d"

== system Y3Tiltrotor_sim3_INDI/Subsystem/固定翼模态/高度-速度控制/定速模式 ==
  Height_d : Inport
  Xe : Inport  Port=2
  Ve : Inport  Port=3
  Manual Vz_d : Inport  Port=4
  Manual : Inport  Port=5
  FW_Airspeed_d : Inport  Port=6
  V_ref : Inport  Port=7
  Airspeed : Inport  Port=8
  gamma : Inport  Port=9
  CoupledControl : Inport  Port=10
  Action Port : ActionPort  ActionPortLabel=case [ 2 ]:
  Subsystem1 : Subsystem
  Switch : Switch  Criteria=u2 > Threshold  SaturateOnIntegerOverflow=off  InputSameDT=off
  Switch1 : Switch  Criteria=u2 > Threshold  SaturateOnIntegerOverflow=off  InputSameDT=off
  TECS : Subsystem
  airspeed control : Subsystem
  Pitch_d_spe : Outport
  Thrust_spe : Outport  Port=2
  wires:
  Height_d/1 -> Subsystem1/3(Height_d), TECS/2(h_d)
  Xe/1 -> TECS/3(Xe), Subsystem1/5(Xe)
  FW_Airspeed_d/1 -> TECS/4(Airspeed_d), airspeed control/2(Airspeed_d)
  Airspeed/1 -> TECS/6(Airspeed), airspeed control/4(Airspeed)
  gamma/1 -> TECS/7(gamma)
  TECS/2(Throttle) -> Switch/1
  CoupledControl/1 -> Switch/2, Switch1/2
  TECS/1(Theta_d) -> Switch1/1
  Switch1/1 -> Pitch_d_spe/1
  Switch/1 -> Thrust_spe/1
  airspeed control/1(Throttle) -> Switch/3
  Subsystem1/1(Pitch_d_alt) -> Switch1/3
  Ve/1 -> Subsystem1/2(Ve)
  Manual Vz_d/1 -> Subsystem1/4(Manual Vz_d)
  Manual/1 -> airspeed control/1(Manual), TECS/1(Manual), Subsystem1/1(Manual)
  V_ref/1 -> airspeed control/3(V_ref), TECS/5(V_ref)

== system Y3Tiltrotor_sim3_INDI/Subsystem/固定翼模态/高度-速度控制/定高模式 ==
  FW_Thrust_sta : Inport
  Manual : Inport  Port=2
  Manual Vz_d : Inport  Port=3
  Ve : Inport  Port=4
  Height_d : Inport  Port=5
  Xe : Inport  Port=6
  Action Port : ActionPort  ActionPortLabel=case [ 1 ]:
  Gain : Gain  Gain=-1
  PID Controller1 : slpidlib/PID Controller  Controller=PID  Form=Parallel  TimeDomain=Continuous-time  UseExternalTs=off  SampleTime=ControlSampleTime  IntegratorMethod=Forward Euler  FilterMethod=Forward Euler  ControllerParametersSource=internal  P=control.FW.vz_P  I=control.FW.vz_I  UseKiTs=off  D=control.FW.vz_D  UseExternalDerivativeSource=off  N=100  UseFilter=on  TunerSelectOption=Transfer Function Based (PID Tuner App)  InitialConditionSource=internal  InitialConditionForIntegrator=0  InitialConditionForFilter=0  DifferentiatorICPrevScaledInput=0  ExternalReset=none  TrackingMode=off  Kt=1  LimitOutput=on  SatLimitsSource=internal  UpperSaturationLimit=control.maxPitch  LowerSaturationLimit=control.minPitch  LinearizeAsGain=on  AntiWindupMode=clamping  Kb=1  LimitIntegrator=off  UpperIntegratorSaturationLimit=inf  LowerIntegratorSaturationLimit=-inf  POutMin=[]  POutMax=[]  IOutMin=[]  IOutMax=[]  DOutMin=[]  DOutMax=[]  NOutMin=[]  NOutMax=[]  SumOutMin=[]  SumOutMax=[]  SaturationOutMin=[]  SaturationOutMax=[]  PParamMin=[]  PParamMax=[]  IParamMin=[]  IParamMax=[]  DParamMin=[]  DParamMax=[]  NParamMin=[]  NParamMax=[]  KbParamMin=[]  KbParamMax=[]  KtParamMin=[]  KtParamMax=[]  KbOutMin=[]  KbOutMax=[]  KtOutMin=[]  KtOutMax=[]  IntegratorOutMin=[]  IntegratorOutMax=[]  FilterOutMin=[]  FilterOutMax=[]  SumI1OutMin=[]  SumI1OutMax=[]  SumI2OutMin=[]  SumI2OutMax=[]  SumI3OutMin=[]  SumI3OutMax=[]  SumI4OutMin=[]  SumI4OutMax=[]  SumDOutMin=[]  SumDOutMax=[]  DifferentiatorOutMin=[]  DifferentiatorOutMax=[]  FilterDiffOutCoefMin=[]  FilterDiffOutCoefMax=[]  ReciprocalOutMin=[]  ReciprocalOutMax=[]  SumDenOutMin=[]  SumDenOutMax=[]  SumNumOutMin=[]  SumNumOutMax=[]  DivideOutMin=[]  DivideOutMax=[]  UdiffTsProdOutMin=[]  UdiffTsProdOutMax=[]  NTsProdOutMin=[]  NTsProdOutMax=[]  UintegralTsProdOutMin=[]  UintegralTsProdOutMax=[]  UngainTsProdOutMin=[]  UngainTsProdOutMax=[]  ClampingZeroOutDataTypeStr=Inherit: Inherit via back propagation  ClampingZeroOutMin=[]  ClampingZeroOutMax=[]  FilterDenConstantOutDataTypeStr=Inherit: Inherit via back propagation  FilterDenConstantOutMin=[]  FilterDenConstantOutMax=[]  PCopyOutDataTypeStr=Inherit: Inherit via back propagation  PCopyOutMin=[]  PCopyOutMax=[]  NCopyOutDataTypeStr=Inherit: Inherit via back propagation  NCopyOutMin=[]  NCopyOutMax=[]  IntegratorContinuousStateAttributes=''  IntegratorStateMustResolveToSignalObject=off  IntegratorRTWStateStorageClass=Auto  FilterContinuousStateAttributes=''  FilterStateMustResolveToSignalObject=off  FilterRTWStateStorageClass=Auto  ParallelPVariant=InternalParameters  IdealPVariant=Disabled  IVariant=InternalParameters  DVariant=InternalParameters  IntegratorVariant=Continuous  SatVariant=Enabled  AWVariant=ContClampingParallel  PCopyVariant=Disabled  TRVariant=Disabled  FdbkBlocksVariant=Forward  IdealPFdbkVariant=Disabled  SatFdbkVariant=Disabled  DerivativeFilterVariant=ContFilter  NVariant=InternalParameters  NCopyVariant=Disabled  FilterICVariant=InternalICsFilter  IntegratorICVariant=InternalICs  ExternalResetVariant=Disabled  TRSumVariant=Passthrough  SumFdbkVariant=Disabled  SumVariant=Sum_PID  TsampFilterVariant=InternalTs  TsampNgainVariant=Passthrough  TsampIntegralVariant=Disabled_SignalSpec  ExternalSaturationOutDataTypeStr=Inherit: Same as second input  DerivativeSourceVariant=ErrorSignal  PreIntVariant=InternalPreInt
  Selector1 : Selector  InputPortWidth=3  IndexOptions=Index vector (dialog)  Indices=3  OutputSizes=1
  Subsystem : Subsystem
  Sum1 : Sum  Inputs=|+-
  Terminator : Terminator
  Transfer Fcn : TransferFcn  Numerator=[5]  Denominator=[1 5]
  Unary Minus1 : UnaryMinus
  Pitch_d_alt : Outport
  Thrust_alt : Outport  Port=2
  wires:
  FW_Thrust_sta/1 -> Thrust_alt/1
  Ve/1 -> Selector1/1
  Sum1/1 -> PID Controller1/1
  Selector1/1 -> Unary Minus1/1
  Gain/1 -> Terminator/1  "Vz_d"
  Transfer Fcn/1 -> Gain/1, Sum1/1
  Unary Minus1/1 -> Sum1/2
  PID Controller1/1 -> Pitch_d_alt/1
  Subsystem/1(Vz_d) -> Transfer Fcn/1
  Manual/1 -> Subsystem/1(Manual)
  Manual Vz_d/1 -> Subsystem/3(Manual Vz_d)
  Xe/1 -> Subsystem/4(Xe)
  Height_d/1 -> Subsystem/2(Height_d)

== system Y3Tiltrotor_sim3_INDI/Subsystem/固定翼模态/高度-速度控制/自稳模式 ==
  FW_Pitch_d_sta : Inport
  FW_Thrust_sta : Inport  Port=2
  Action Port : ActionPort  ActionPortLabel=case [ 0 ]:
  Pitch_d_sta : Outport
  Thrust_sta : Outport  Port=2
  wires:
  FW_Pitch_d_sta/1 -> Pitch_d_sta/1
  FW_Thrust_sta/1 -> Thrust_sta/1

== system Y3Tiltrotor_sim3_INDI/Subsystem/多旋翼模态/Multirotor XY control/Subsystem ==
  y : Inport
  Manual : Inport  Port=2
  Ch2 : Inport  Port=3
  y_ref : Inport  Port=4
  InputConditioning_altitude : Subsystem
  Merge : Merge
  Subsystem : Subsystem
  Switch Case : SwitchCase  CaseConditions={0,1}  ShowDefaultCase=off
  MR_vy_d : Outport
  wires:
  Ch2/1 -> InputConditioning_altitude/1(Ch2)
  InputConditioning_altitude/1(manual_vlat_cmd) -> Merge/2  "Manual vy_d"
  Manual/1 -> Switch Case/1
  Switch Case/2 -> InputConditioning_altitude/Action
  Subsystem/1(PID_vy_cmd) -> Merge/1  "PID_vy_d"
  Switch Case/1 -> Subsystem/Action
  Merge/1 -> MR_vy_d/1
  y_ref/1 -> Subsystem/1(y_ref)
  y/1 -> Subsystem/2(y)

== system Y3Tiltrotor_sim3_INDI/Subsystem/多旋翼模态/Multirotor XY control/Subsystem3 ==
  Manual : Inport
  Ch8 : Inport  Port=2
  x_ref : Inport  Port=3
  x : Inport  Port=4
  InputConditioning_altitude : Subsystem
  Merge : Merge
  Subsystem : Subsystem
  Switch Case : SwitchCase  CaseConditions={0,1}  ShowDefaultCase=off
  MR_vx_d : Outport
  wires:
  Merge/1 -> MR_vx_d/1
  Switch Case/1 -> Subsystem/Action
  Subsystem/1(PID_vx_cmd) -> Merge/1  "PID_vx_d"
  Switch Case/2 -> InputConditioning_altitude/Action
  Manual/1 -> Switch Case/1
  InputConditioning_altitude/1(manual_vfor_cmd) -> Merge/2  "Manual vx_d"
  Ch8/1 -> InputConditioning_altitude/1(Ch8)
  x_ref/1 -> Subsystem/1(x_ref)
  x/1 -> Subsystem/2(x)

== system Y3Tiltrotor_sim3_INDI/Subsystem/多旋翼模态/Multirotor altitude control/Subsystem ==
  Manual : Inport
  Ch3 : Inport  Port=2
  Xe : Inport  Port=3
  z_ref : Inport  Port=4
  Gain : Gain  Gain=-1
  InputConditioning_altitude : Subsystem
  Merge : Merge
  Selector : Selector  InputPortWidth=3  IndexOptions=Index vector (dialog)  Indices=3  OutputSizes=1
  Subsystem : Subsystem
  Switch Case : SwitchCase  CaseConditions={0,1}  ShowDefaultCase=off
  vz_d : Outport
  wires:
  Ch3/1 -> InputConditioning_altitude/1(Ch3)
  Xe/1 -> Selector/1, InputConditioning_altitude/2(Xe)
  InputConditioning_altitude/1(Manual vz_d) -> Merge/2  "Manual vz_d"
  Manual/1 -> Switch Case/1
  Switch Case/2 -> InputConditioning_altitude/Action
  Subsystem/1(PID_vz_cmd) -> Merge/1  "PID vz_d"
  Switch Case/1 -> Subsystem/Action
  Merge/1 -> vz_d/1
  z_ref/1 -> Subsystem/1(z_ref)
  Selector/1 -> Gain/1
  Gain/1 -> Subsystem/2(z)

== system Y3Tiltrotor_sim3_INDI/Subsystem/多旋翼模态/Multirotor attitude control (INDI)/INDI in vector form ==
  pqr_d : Inport
  pqr : Inport  Port=2
  Demux : Demux  Outputs=3
  Derivative1 : Derivative
  Derivative2 : Derivative
  Gain1 : Gain  Gain=[k_p 0 0;0 k_q 0;0 0 k_r]  Multiplication=Matrix(K*u) (u vector)
  Gain2 : Gain  Gain=[uavParam.inertia.Ixx 0 0;0 uavParam.inertia.Iyy 0;0 0 uavParam.inertia.Izz]  Multiplication=Matrix(K*u) (u vector)
  Gain3 : Gain  Gain=1/(9.5883e-7*1.225*pi*0.765^4*(19741.896106*2*pi/60)^2)
  Mux : Mux  Inputs=3
  Subsystem : Subsystem
  Subsystem1 : Subsystem
  Subsystem2 : Subsystem
  Sum : Sum  Inputs=|++
  Sum1 : Sum  Inputs=|+-
  Sum2 : Sum  Inputs=++-
  p_测量噪声 : Subsystem
  q_测量噪声 : Subsystem
  r_测量噪声 : Subsystem
  u_pqr : Outport
  wires:
  pqr_d/1 -> Sum1/1, Derivative1/1
  Sum1/1 -> Gain1/1  "e_pqr_INDI"
  Sum2/1 -> Gain2/1
  Gain2/1 -> Gain3/1
  Gain1/1 -> Sum2/2
  Derivative2/1 -> Subsystem1/1(original)
  Subsystem1/1(LPF) -> Sum2/3
  Derivative1/1 -> Subsystem/1(original)
  Subsystem/1(LPF) -> Sum2/1
  Gain3/1 -> Sum/1
  Sum/1 -> Subsystem2/1(original), u_pqr/1
  Subsystem2/1(LPF) -> Sum/2
  pqr/1 -> Demux/1
  Mux/1 -> Sum1/2, Derivative2/1
  Demux/3 -> Mux/3
  Demux/2 -> Mux/2
  Demux/1 -> Mux/1

== system Y3Tiltrotor_sim3_INDI/Subsystem/多旋翼模态/Multirotor attitude control (INDI)/INDI_p ==
  MR_p_d : Inport
  p : Inport  Port=2
  Derivative : Derivative
  Derivative1 : Derivative
  Gain : Gain  Gain=uavParam.inertia.Ixx/(9.5883e-7*1.225*pi*0.765^4*(19741.896106*2*pi/60)^2)
  Gain1 : Gain  Gain=k_p
  Memory : Memory
  Sum : Sum  Inputs=|++
  Sum1 : Sum  Inputs=|+-
  Sum2 : Sum  Inputs=++-
  Transfer Fcn3 : TransferFcn  Numerator=[k_lpf_p]  Denominator=[1 k_lpf_p]
  Transfer Fcn4 : TransferFcn  Numerator=[k_lpf_p]  Denominator=[1 k_lpf_p]
  Transfer Fcn7 : TransferFcn  Numerator=[k_lpf_p]  Denominator=[1 k_lpf_p]
  u_roll : Outport
  wires:
  MR_p_d/1 -> Derivative1/1, Sum1/1
  Gain/1 -> Sum/1
  Sum2/1 -> Gain/1
  Sum1/1 -> Gain1/1
  Gain1/1 -> Sum2/2
  Sum/1 -> Transfer Fcn7/1, u_roll/1
  p/1 -> Derivative/1, Sum1/2
  Transfer Fcn7/1 -> Sum/2
  Transfer Fcn4/1 -> Sum2/3  "p_dot_0"
  Derivative1/1 -> Transfer Fcn3/1
  Transfer Fcn3/1 -> Sum2/1  "p_d_dot"
  Derivative/1 -> Transfer Fcn4/1

== system Y3Tiltrotor_sim3_INDI/Subsystem/多旋翼模态/Multirotor attitude control (INDI)/INDI_q ==
  MR_q_d : Inport
  q : Inport  Port=2
  Derivative : Derivative
  Derivative1 : Derivative
  Gain : Gain  Gain=uavParam.inertia.Iyy/(9.5883e-7*1.225*pi*0.765^4*(19741.896106*2*pi/60)^2)
  Gain1 : Gain  Gain=k_q
  Sum : Sum  Inputs=|++
  Sum1 : Sum  Inputs=|+-
  Sum2 : Sum  Inputs=++-
  Transfer Fcn3 : TransferFcn  Numerator=[k_lpf_q]  Denominator=[1 k_lpf_q]
  Transfer Fcn4 : TransferFcn  Numerator=[k_lpf_q]  Denominator=[1 k_lpf_q]
  Transfer Fcn7 : TransferFcn  Numerator=[k_lpf_q]  Denominator=[1 k_lpf_q]
  u_theta : Outport
  wires:
  MR_q_d/1 -> Derivative1/1, Sum1/1
  Gain/1 -> Sum/1
  Sum2/1 -> Gain/1
  Derivative1/1 -> Transfer Fcn3/1  "q_d_dot"
  Sum1/1 -> Gain1/1
  Gain1/1 -> Sum2/2
  Sum/1 -> Transfer Fcn7/1, u_theta/1
  q/1 -> Derivative/1, Sum1/2
  Derivative/1 -> Transfer Fcn4/1
  Transfer Fcn3/1 -> Sum2/1
  Transfer Fcn4/1 -> Sum2/3  "q_dot_0"
  Transfer Fcn7/1 -> Sum/2

== system Y3Tiltrotor_sim3_INDI/Subsystem/多旋翼模态/Multirotor attitude control (INDI)/INDI_r ==
  MR_r_d : Inport
  r : Inport  Port=2
  Derivative : Derivative
  Derivative1 : Derivative
  Gain : Gain  Gain=uavParam.inertia.Izz/(9.5883e-7*1.225*pi*0.765^4*(19741.896106*2*pi/60)^2)
  Gain1 : Gain  Gain=k_r
  Sum : Sum  Inputs=|++
  Sum1 : Sum  Inputs=|+-
  Sum2 : Sum  Inputs=++-
  Transfer Fcn3 : TransferFcn  Numerator=[k_lpf_r]  Denominator=[1 k_lpf_r]
  Transfer Fcn4 : TransferFcn  Numerator=[k_lpf_r]  Denominator=[1 k_lpf_r]
  Transfer Fcn7 : TransferFcn  Numerator=[k_lpf_r]  Denominator=[1 k_lpf_r]
  u_psi : Outport
  wires:
  Transfer Fcn7/1 -> Sum/2
  Transfer Fcn4/1 -> Sum2/3  "r_dot_0"
  Transfer Fcn3/1 -> Sum2/1
  Derivative/1 -> Transfer Fcn4/1
  r/1 -> Sum1/2, Derivative/1
  Sum/1 -> u_psi/1, Transfer Fcn7/1
  Gain1/1 -> Sum2/2
  Sum1/1 -> Gain1/1
  Derivative1/1 -> Transfer Fcn3/1  "r_d_dot"
  Sum2/1 -> Gain/1
  Gain/1 -> Sum/1
  MR_r_d/1 -> Sum1/1, Derivative1/1

== system Y3Tiltrotor_sim3_INDI/Subsystem/多旋翼模态/Multirotor attitude control (INDI)/Subsystem ==
  Manual : Inport
  Euler_d : Inport  Port=2
  Euler : Inport  Port=3
  YawRate_d : Inport  Port=4
  YawRate : Inport  Port=5
  Merge : Merge
  Selector1 : Selector  InputPortWidth=3  IndexOptions=Index vector (dialog)  Indices=3  OutputSizes=1
  Selector7 : Selector  InputPortWidth=3  IndexOptions=Index vector (dialog)  Indices=3  OutputSizes=1
  Subsystem : Subsystem
  Subsystem1 : Subsystem
  Switch Case : SwitchCase  CaseConditions={0,1}  ShowDefaultCase=off
  MR_r_d : Outport
  wires:
  Merge/1 -> MR_r_d/1
  Manual/1 -> Switch Case/1
  Euler_d/1 -> Subsystem/1(Euler_d)
  Euler/1 -> Subsystem/2(Euler), Selector1/1
  Subsystem/1(MR_r_d) -> Merge/1
  YawRate_d/1 -> Subsystem1/1(YawRate_d)
  Subsystem1/1(r_d) -> Merge/2
  Switch Case/2 -> Subsystem1/Action
  Switch Case/1 -> Subsystem/Action
  Selector7/1 -> Subsystem1/3(YawRate)
  YawRate/1 -> Selector7/1
  Selector1/1 -> Subsystem1/2(Yaw)

== system Y3Tiltrotor_sim3_INDI/Subsystem/多旋翼模态/Velocity Control/INDI in vector form ==
  uvw_d : Inport
  uvw : Inport  Port=2
  Derivative1 : Derivative
  Derivative2 : Derivative
  Gain1 : Gain  Gain=[k_u 0 0;0 k_v 0;0 0 k_w]  Multiplication=Matrix(K*u) (u vector)
  Gain2 : Gain  Gain=[uavParam.geom.mass/(9.5883e-7*1.225*pi*0.765^4*(19741.896106*2*pi/60)^2) 0 0;0 uavParam.geom.mass 0;0 0 uavParam.geom.mass/(9.5883e-7*1.225*pi*0.765^4*(19741.896106*2*pi/60)^2)]  Multiplication=Matrix(K*u) (u vector)
  Subsystem1 : Subsystem
  Subsystem3 : Subsystem
  Sum : Sum  Inputs=|++
  Sum1 : Sum  Inputs=|+-
  Sum2 : Sum  Inputs=++-
  u_uvw : Outport
  wires:
  uvw_d/1 -> Sum1/1, Derivative1/1
  uvw/1 -> Derivative2/1, Sum1/2
  Sum1/1 -> Gain1/1  "e_uvw_INDI"
  Sum2/1 -> Gain2/1
  Gain1/1 -> Sum2/2
  Derivative2/1 -> Subsystem1/1(original)
  Subsystem1/1(LPF) -> Sum2/3
  Derivative1/1 -> Sum2/1
  Gain2/1 -> Sum/1
  Sum/1 -> Subsystem3/1(original), u_uvw/1
  Subsystem3/1(LPF) -> Sum/2

== system Y3Tiltrotor_sim3_INDI/Subsystem/多旋翼模态/Velocity Control/INDI_u ==
  MR_u_d : Inport
  u : Inport  Port=2
  Derivative : Derivative
  Derivative1 : Derivative
  Gain : Gain  Gain=uavParam.geom.mass/(9.5883e-7*1.225*pi*0.765^4*(19741.896106*2*pi/60)^2)
  Gain1 : Gain  Gain=k_u
  Sum : Sum  Inputs=|++
  Sum1 : Sum  Inputs=|+-
  Sum2 : Sum  Inputs=++-
  Transfer Fcn3 : TransferFcn  Numerator=[k_lpf_u]  Denominator=[1 k_lpf_u]
  Transfer Fcn4 : TransferFcn  Numerator=[k_lpf_u]  Denominator=[1 k_lpf_u]
  Transfer Fcn7 : TransferFcn  Numerator=[k_lpf_u]  Denominator=[1 k_lpf_u]
  u_u : Outport
  wires:
  Transfer Fcn4/1 -> Sum2/3  "u_dot_0"
  Derivative/1 -> Transfer Fcn4/1
  Derivative1/1 -> Sum2/1  "u_d_dot"
  MR_u_d/1 -> Derivative1/1, Sum1/1
  Gain/1 -> Sum/1
  Sum2/1 -> Gain/1
  Sum1/1 -> Gain1/1  "e_u_INDI"
  Gain1/1 -> Sum2/2
  Sum/1 -> u_u/1, Transfer Fcn7/1
  u/1 -> Derivative/1, Sum1/2
  Transfer Fcn7/1 -> Sum/2

== system Y3Tiltrotor_sim3_INDI/Subsystem/多旋翼模态/Velocity Control/INDI_v ==
  MR_v_d : Inport
  v : Inport  Port=2
  Derivative : Derivative
  Derivative1 : Derivative
  Gain : Gain  Gain=uavParam.geom.mass
  Gain1 : Gain  Gain=k_v
  Sum : Sum  Inputs=|++
  Sum1 : Sum  Inputs=|+-
  Sum2 : Sum  Inputs=++-
  Transfer Fcn3 : TransferFcn  Numerator=[k_lpf_v]  Denominator=[1 k_lpf_v]
  Transfer Fcn4 : TransferFcn  Numerator=[k_lpf_v]  Denominator=[1 k_lpf_v]
  Transfer Fcn7 : TransferFcn  Numerator=[k_lpf_v]  Denominator=[1 k_lpf_v]
  u_v : Outport
  wires:
  Transfer Fcn7/1 -> Sum/2
  v/1 -> Sum1/2, Derivative/1
  Sum/1 -> Transfer Fcn7/1, u_v/1
  Gain1/1 -> Sum2/2
  Sum1/1 -> Gain1/1  "e_v_INDI"
  Sum2/1 -> Gain/1
  Gain/1 -> Sum/1
  MR_v_d/1 -> Sum1/1, Derivative1/1
  Derivative1/1 -> Sum2/1  "v_d_dot"
  Derivative/1 -> Transfer Fcn4/1
  Transfer Fcn4/1 -> Sum2/3  "v_dot_0"

== system Y3Tiltrotor_sim3_INDI/Subsystem/多旋翼模态/Velocity Control/INDI_w ==
  MR_w_d : Inport
  w : Inport  Port=2
  Derivative : Derivative
  Derivative1 : Derivative
  Gain : Gain  Gain=uavParam.geom.mass/(9.5883e-7*1.225*pi*0.765^4*(19741.896106*2*pi/60)^2)
  Gain1 : Gain  Gain=k_w
  Sum : Sum  Inputs=|++
  Sum1 : Sum  Inputs=|+-
  Sum2 : Sum  Inputs=++-
  Transfer Fcn3 : TransferFcn  Numerator=[k_lpf_w]  Denominator=[1 k_lpf_w]
  Transfer Fcn4 : TransferFcn  Numerator=[k_lpf_w]  Denominator=[1 k_lpf_w]
  Transfer Fcn7 : TransferFcn  Numerator=[k_lpf_w]  Denominator=[1 k_lpf_w]
  u_w : Outport
  wires:
  MR_w_d/1 -> Derivative1/1, Sum1/1
  Gain/1 -> Sum/1
  Sum2/1 -> Gain/1
  Sum1/1 -> Gain1/1  "e_w_INDI"
  Gain1/1 -> Sum2/2
  Sum/1 -> Transfer Fcn7/1, u_w/1
  w/1 -> Derivative/1, Sum1/2
  Transfer Fcn7/1 -> Sum/2
  Transfer Fcn4/1 -> Sum2/3  "w_dot_0"
  Derivative/1 -> Transfer Fcn4/1
  Derivative1/1 -> Sum2/1  "w_d_dot"
